simulink model "hrg_wa_a1_port_deembedding"  (R2025a)
settings: Solver=ode113  StartTime=0.0  StopTime=.04  MaxStep=1/200000  RelTol=1e-10  AbsTol=1e-12
settings Model: Creator=11725  LastModifiedBy=11725

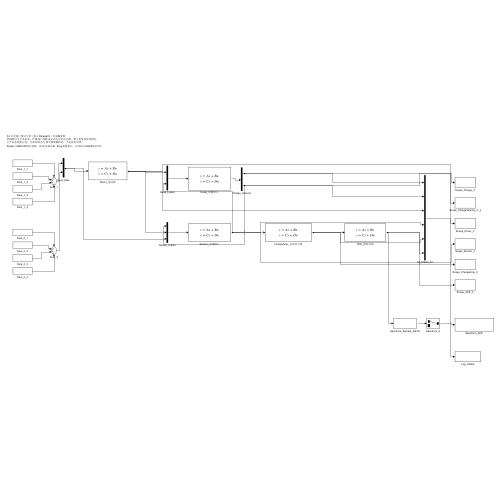
[thumbnail: Simulink's stored preview of the top-level diagram]
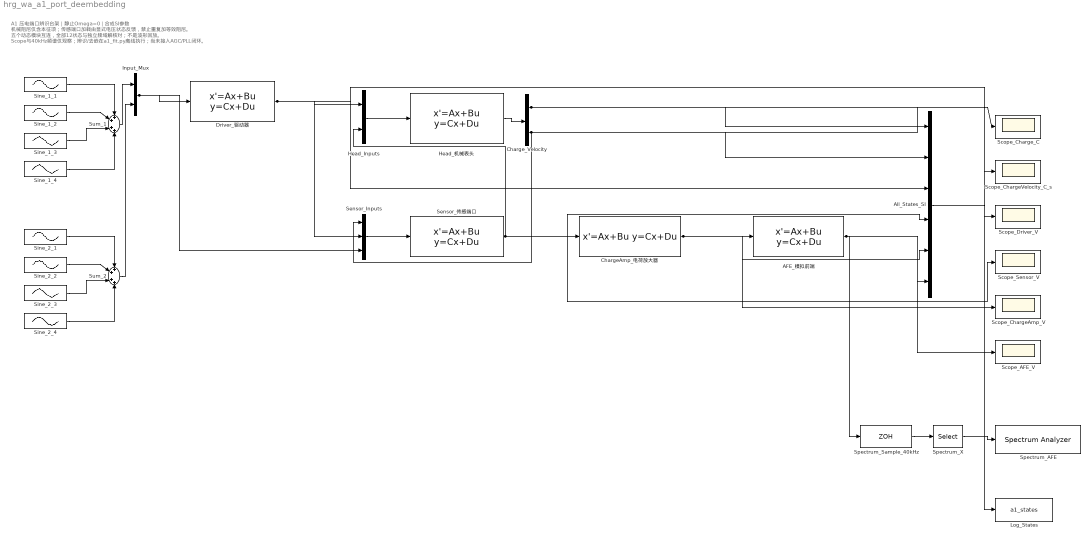
== system hrg_wa_a1_port_deembedding ==
  note: A1 压电端口辨识台架｜静止Omega=0｜合成SI参数
      | 机械阻尼仅含本征项；传感端口加载由显式电压状态反馈，禁止重复加等效阻尼。
      | 五个动态模块互连，全部12状态与独立频域解核对；不是波形回放。
      | Scope与40kHz频谱仅观察；辨识/去嵌在a1_fit.py离线执行；尚未接入AGC/PLL闭环。
  AFE_模拟前端 : StateSpace  A=[-28274.333882308139 0;0 -21991.148575128551]  B=[339594.61051325151 24705.197173591092;-15838.148980526914 190378.76810432039]  C=[0.099999999999999992 0;0 0.099999999999999992]  D=[0 0;0 0]  InitialCondition=[-0.011179243937679948;-0.0061390962673901301]
  All_States_SI : Mux  Inputs=6
  ChargeAmp_电荷放大器 : StateSpace  A=[-10 0;0 -10]  B=[1250000 0;0 1250000]  C=[0.099999999999999992 0;0 0.099999999999999992]  D=[0 0;0 0]  InitialCondition=[-0.0091848117130703746;-0.0068852582734945829]
  Charge_Velocity : Demux  Outputs=[2 2]
  Driver_驱动器 : StateSpace  A=[-49999.999999999993 0;0 -41666.666666666664]  B=[49999.999999999993 0;0 41666.666666666664]  C=[1 0;0 1]  D=[0 0;0 0]  InitialCondition=[0.032649927053302302;0.0076946539687300563]
  Head_Inputs : Mux  Inputs=2
  Head_机械表头 : StateSpace  A=[0 0 6283.1853071795849 0;0 0 0 6283.1853071795849;-6281.7934681118495 1.2710027697449111 -0.77168693032204283 0.071031697114483178;1.2710027697449111 -6284.5774289906631 0.071031697114483178 -0.48495013111387464]  B=[0 0 0 0;0 0 0 0;17.393903554643085 -0.36204154460282534 15.915494309189537 0;0.50627845929276083 18.638783902499984 0 15.915494309189537]  C=[9.9999999999999994e-12 0 0 0;0 9.9999999999999994e-12 0 0;0 0 6.2831853071795849e-08 0;0 0 0 6.2831853071795849e-08]  D=[0 0 0 0;0 0 0 0;0 0 0 0;0 0 0 0]  InitialCondition=[0.0092134405690375114;0.0041850616558849257;-0.0045197077257580218;-0.0088226761833289126]
  Input_Mux : Mux  Inputs=2
  Log_States : ToWorkspace  VariableName=a1_states  SaveFormat=Timeseries  SampleTime=-1
  Scope_AFE_V : Scope
  Scope_ChargeAmp_V : Scope
  Scope_ChargeVelocity_C_s : Scope
  Scope_Charge_C : Scope
  Scope_Driver_V : Scope
  Scope_Sensor_V : Scope
  Sensor_Inputs : Mux  Inputs=3
  Sensor_传感端口 : StateSpace  A=[-12500.1 0;0 -12500.1]  B=[-198943678864.8692 0 0 0 0 0;0 -198943678864.8692 0 0 0 0]  C=[0.0050265482457436681 0;0 0.0050265482457436681]  D=[0 0 0 0 0 0;0 0 0 0 0 0]  InitialCondition=[-5.6951115084558776e-05;0.0053892373995855425]
  Sine_1_1 : Sin  Amplitude=0.01  Frequency=3769.9111843077517  Phase=1.8707963267948964  SampleTime=0
  Sine_1_2 : Sin  Amplitude=0.01  Frequency=6273.7605292188173  Phase=2.1707963267948966  SampleTime=0
  Sine_1_3 : Sin  Amplitude=0.01  Frequency=8796.45943005142  Phase=2.4707963267948965  SampleTime=0
  Sine_1_4 : Sin  Amplitude=0.01  Frequency=40840.704496667313  Phase=2.7707963267948967  SampleTime=0
  Sine_2_1 : Sin  Amplitude=0.01  Frequency=3769.9111843077517  Phase=2.3407963267948966  SampleTime=0
  Sine_2_2 : Sin  Amplitude=0.01  Frequency=6273.7605292188173  Phase=2.9407963267948967  SampleTime=0
  Sine_2_3 : Sin  Amplitude=0.01  Frequency=8796.45943005142  Phase=3.5407963267948963  SampleTime=0
  Sine_2_4 : Sin  Amplitude=0.01  Frequency=40840.704496667313  Phase=4.1407963267948968  SampleTime=0
  Spectrum_AFE : SpectrumAnalyzer  SampleRateSource=Property  SampleRate=40000  WindowInvariantSamplesPerUpdate=on  SpectrumUnits=dBV
      settings: OpenAtSimulationStart=off
  Spectrum_Sample_40kHz : ZeroOrderHold  SampleTime=1/40000
  Spectrum_X : Selector  InputPortWidth=2  IndexOptions=Index vector (dialog)  Indices=1  OutputSizes=1
  Sum_1 : Sum  Inputs=++++
  Sum_2 : Sum  Inputs=++++
  wires:
  Sine_1_1/1 -> Sum_1/1
  Sine_1_2/1 -> Sum_1/2
  Sine_1_3/1 -> Sum_1/3
  Sine_1_4/1 -> Sum_1/4
  Sum_1/1 -> Input_Mux/1
  Sine_2_1/1 -> Sum_2/1
  Sine_2_2/1 -> Sum_2/2
  Sine_2_3/1 -> Sum_2/3
  Sine_2_4/1 -> Sum_2/4
  Sum_2/1 -> Input_Mux/2
  Input_Mux/1 -> Driver_驱动器/1, Sensor_Inputs/3
  Driver_驱动器/1 -> Head_Inputs/1, Sensor_Inputs/2, All_States_SI/3, Scope_Driver_V/1
  Sensor_传感端口/1 -> Head_Inputs/2, ChargeAmp_电荷放大器/1, All_States_SI/4, Scope_Sensor_V/1
  Head_Inputs/1 -> Head_机械表头/1
  Head_机械表头/1 -> Charge_Velocity/1
  Charge_Velocity/2 -> Sensor_Inputs/1, All_States_SI/2, Scope_ChargeVelocity_C_s/1
  Sensor_Inputs/1 -> Sensor_传感端口/1
  ChargeAmp_电荷放大器/1 -> AFE_模拟前端/1, All_States_SI/5, Scope_ChargeAmp_V/1
  Charge_Velocity/1 -> All_States_SI/1, Scope_Charge_C/1
  AFE_模拟前端/1 -> All_States_SI/6, Scope_AFE_V/1, Spectrum_Sample_40kHz/1
  All_States_SI/1 -> Log_States/1
  Spectrum_Sample_40kHz/1 -> Spectrum_X/1
  Spectrum_X/1 -> Spectrum_AFE/1
